simulink subsystem "tui_debug_state_publisher"  (R2026a)
settings: Solver=VariableStepAuto
undefined symbols (not defined in the file): S
libraries: ros2lib x2
settings Model: Creator=kjhaydon  LastModifiedBy=kjhaydon

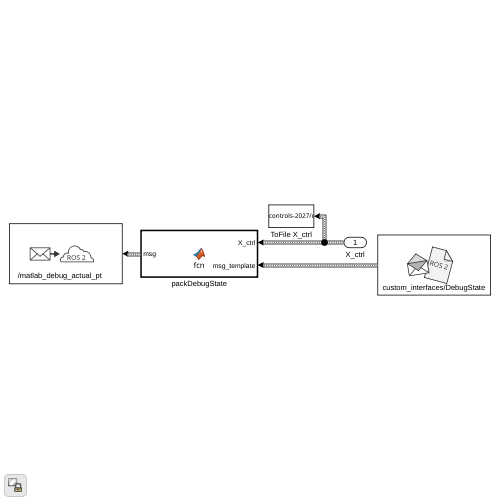
[thumbnail: Simulink's stored preview of the top-level diagram]
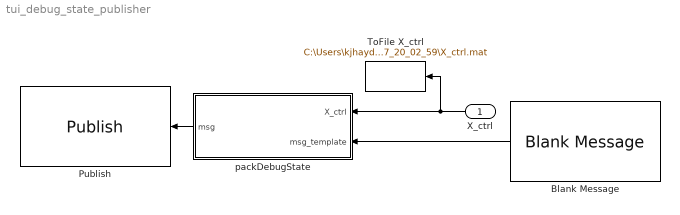
== system tui_debug_state_publisher ==
  X_ctrl : Inport
  Blank Message : ros2lib/Blank Message  messageClass=Message  entityType=custom_interfaces/DebugState  messageType=custom_interfaces/DebugState  SampleTime=inf
  Publish : ros2lib/Publish  topicSource=Specify your own  topic=/matlab_debug_actual_pt  messageType=custom_interfaces/DebugState  QOSHistory=Keep last  QOSDepth=10  QOSReliability=Reliable  QOSDurability=Volatile  QOSDeadline=Inf  QOSLifespan=Inf  QOSLiveliness=Automatic  QOSLeaseDuration=Inf  QOSAvoidROSNamespaceConventions=off
  ToFile X_ctrl : ToFile  Filename=C:\Users\kjhaydon\Documents\GitHub\controls-2027\data\2026_11_17_20_02_59\X_ctrl.mat  MatrixName=X_ctrl  SaveFormat=Timeseries  SampleTime=S.dt_data
  packDebugState : MATLAB Function  TreatAsAtomicUnit=on
  wires:
  Blank Message/1 -> packDebugState/2(msg_template)
  packDebugState/1(msg) -> Publish/1
  X_ctrl/1 -> packDebugState/1(X_ctrl), ToFile X_ctrl/1

== matlab function tui_debug_state_publisher/packDebugState ==
  data: X_ctrl input Bus: X_bus; msg output Bus: SL_Bus_custom_interfaces_DebugState; msg_template input Bus: SL_Bus_custom_interfaces_DebugState
function msg = fcn(X_ctrl, msg_template)

msg = msg_template;

msg.position.x = X_ctrl.Ri(1);
msg.position.y = X_ctrl.Ri(2);
msg.position.z = X_ctrl.Ri(3);
msg.orientation.x = X_ctrl.Eul(1);
msg.orientation.y = X_ctrl.Eul(2);
msg.orientation.z = X_ctrl.Eul(3);
msg.velocity.x = X_ctrl.dRb(1);
msg.velocity.y = X_ctrl.dRb(2);
msg.velocity.z = X_ctrl.dRb(3);
msg.angular_velocity.x = X_ctrl.wb(1); 
msg.angular_velocity.y = X_ctrl.wb(2);
msg.angular_velocity.z = X_ctrl.wb(3);
